simulink model "cbs"  (R2023b)
settings: Solver=FixedStepDiscrete  StartTime=0.0  StopTime=(N-1)*Tb  FixedStep=Tb  RelTol=1e-3
values from neighbouring files (symbols this model uses):
  graine = P.graine    [parametres.m]    (also in parametres_perso.m = mod(sum(c .* (1:numel(c)) * 31) + 7 * numel(c), 2^31 - 1); partie2_1.m)
  p1 = P.p1    [parametres.m]    (also in partie2_1.m; partie2_4_q9.m = mean(bits))
  pe = P.pe_cbs    [parametres.m]    (also in partie2_1.m)
  Tb = 1    [parametres.m]    (also in partie2_1.m)
libraries: simulink x2
settings Model: Creator=e2507477  LastModifiedBy=e2507477

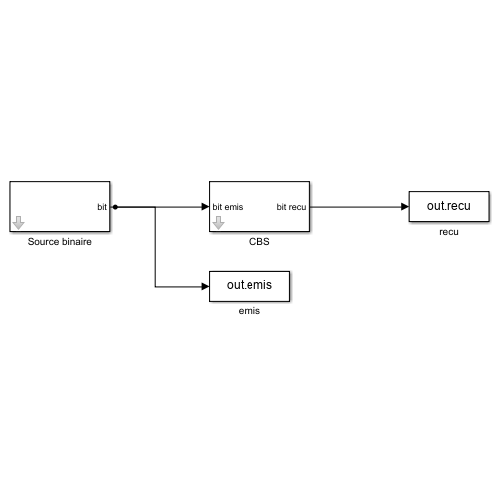
[thumbnail: Simulink's stored preview of the top-level diagram]
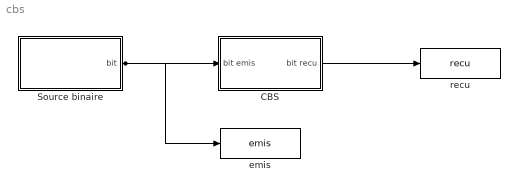
== system cbs ==
  CBS : Subsystem  mask{pe=pe, Tb=Tb, graine=graine}
      mask prompts: pe "Probabilité d'erreur pe"; Tb "Durée d'un bit Tb"
  Source binaire : Subsystem  mask{p1=p1, Tb=Tb, graine=graine}
      mask prompts: p1 "Probabilité d'émettre un 1"; Tb "Durée d'un bit Tb"
  emis : ToWorkspace  VariableName=emis  SampleTime=-1
  recu : ToWorkspace  VariableName=recu  SampleTime=-1
  wires:
  Source binaire/1(bit) -> CBS/1(bit emis), emis/1
  CBS/1(bit recu) -> recu/1

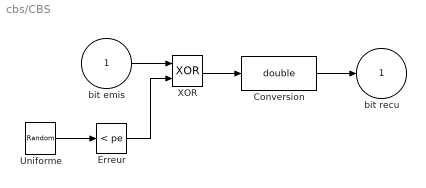
== system cbs/CBS ==
  bit emis : Inport
  Conversion : DataTypeConversion  OutDataTypeStr=double  SaturateOnIntegerOverflow=off  RndMeth=Floor
  Erreur : simulink/Logic and Bit Operations/Compare To Constant  relop=<  const=pe  OutDataTypeStr=boolean
  Uniforme : UniformRandomNumber  Minimum=0  Seed=graine+1  SampleTime=Tb
  XOR : Logic  Operator=XOR  AllPortsSameDT=off  OutDataTypeStr=boolean
  bit recu : Outport
  wires:
  Uniforme/1 -> Erreur/1
  bit emis/1 -> XOR/1
  Erreur/1 -> XOR/2
  Conversion/1 -> bit recu/1
  XOR/1 -> Conversion/1

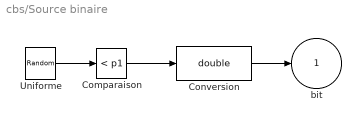
== system cbs/Source binaire ==
  Comparaison : simulink/Logic and Bit Operations/Compare To Constant  relop=<  const=p1  OutDataTypeStr=boolean
  Conversion : DataTypeConversion  OutDataTypeStr=double  SaturateOnIntegerOverflow=off  RndMeth=Floor
  Uniforme : UniformRandomNumber  Minimum=0  Seed=graine  SampleTime=Tb
  bit : Outport
  wires:
  Uniforme/1 -> Comparaison/1
  Comparaison/1 -> Conversion/1
  Conversion/1 -> bit/1
